simulink model "System_Modelled_SIMULINK"  (R2026a)
settings: Solver=VariableStepAuto  StopTime=3600
model workspace (MAT data in the model file):
  T_boot_threshold = 5
  T_overheat = 45
  T_storage_min = 8
  T_target = 15
libraries: fl_lib x12, nesl_utility x7, SignalEditorBlockLib x1

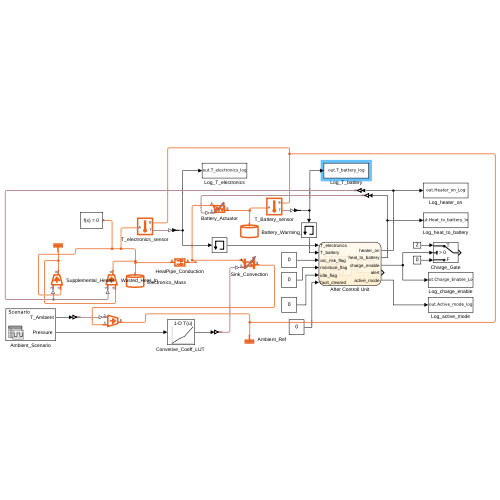
[thumbnail: Simulink's stored preview of the top-level diagram]
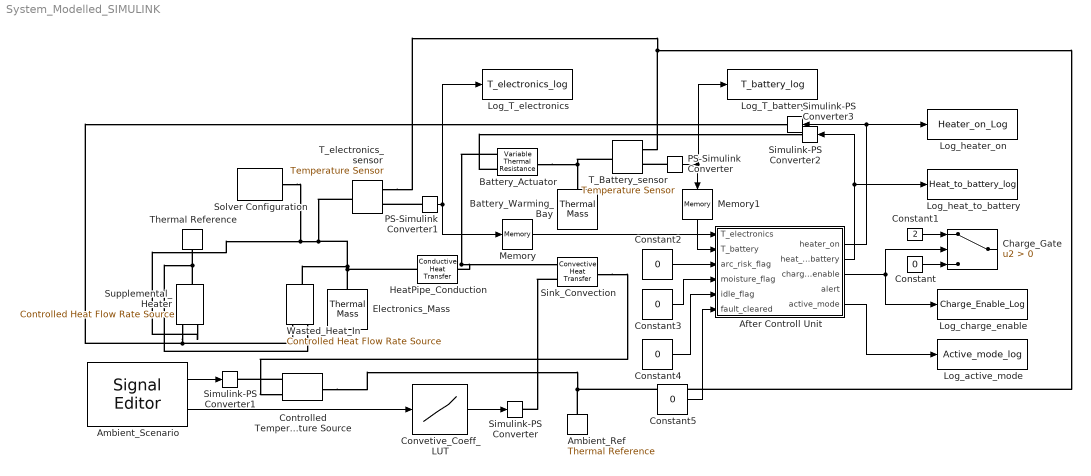
== system System_Modelled_SIMULINK ==
  After Controll Unit : Stateflow chart  TreatAsAtomicUnit=on
  Ambient_Ref : fl_lib/Thermal/Thermal Elements/Thermal Reference
  Ambient_Scenario : SignalEditorBlockLib/Signal Editor  FileName=/MATLAB Drive/SIH/Ambient_Scenario.mat  ActiveScenario=Scenario  ActiveSignal=T_Ambient  IsBus=off  OutputBusObjectStr=Bus: BusObject  SampleTime=0  ZeroCross=off  OutputAfterFinalValue=Setting to zero  Unit=inherit  PreserveSignalName=on  ApplySigPropsToAllScenarios=on  ApplySigPropsToAllSignals=off  SignalPropertySource=Dialog parameters
  Battery_Actuator : fl_lib/Thermal/Thermal Elements/Variable Thermal Resistance  R_min=0 K/W  T_specify=off  T_priority=None  T=0 K  T_nominal_specify=off  T_nominal_value=1  T_nominal_unit=K  Q_specify=off  Q_priority=None  Q=0 W  Q_nominal_specify=off  Q_nominal_value=1  Q_nominal_unit=W
  Battery_Warming_Bay : fl_lib/Thermal/Thermal Elements/Thermal Mass  mass_type=foundation.enum.constant_variable.constant  mass=1 kg  sp_heat=1000 J/(K*kg)  mass_min=1e-6 kg  num_ports=foundation.enum.numPorts2.one  m_specify=off  m_priority=High  m=1 kg  m_nominal_specify=off  m_nominal_value=1  m_nominal_unit=kg  T_specify=off  T_priority=High  T=300 K  T_nominal_specify=off  T_nominal_value=1  T_nominal_unit=K  Q_specify=off  Q_priority=None  Q=0 W  Q_nominal_specify=off  Q_nominal_value=1  Q_nominal_unit=W
  Charge_Gate : Switch  Criteria=u2 > Threshold  SaturateOnIntegerOverflow=off  InputSameDT=off
  Constant{,2..5} (5 alike) : Constant  Value=0
  Constant1 : Constant  Value=2
  Controlled Temperature Source : fl_lib/Thermal/Thermal Sources/Controlled Temperature Source
  "Convetive_Coeff_LUT " : Lookup_n-D  NumberOfTableDimensions=1  BreakpointsForDimension1=[50 60 70 80 101.3]  Table=[3 4 5 6 10]  InternalRulePriority=Speed  RndMeth=Simplest
  Electronics_Mass : fl_lib/Thermal/Thermal Elements/Thermal Mass  mass_type=foundation.enum.constant_variable.constant  mass=3 kg  sp_heat=900 J/(K*kg)  mass_min=1e-6 kg  num_ports=foundation.enum.numPorts2.one  m_specify=off  m_priority=High  m=1 kg  m_nominal_specify=off  m_nominal_value=1  m_nominal_unit=kg  T_specify=off  T_priority=High  T=300 K  T_nominal_specify=off  T_nominal_value=1  T_nominal_unit=K  Q_specify=off  Q_priority=None  Q=0 W  Q_nominal_specify=off  Q_nominal_value=1  Q_nominal_unit=W
  HeatPipe_Conduction : fl_lib/Thermal/Thermal Elements/Conductive Heat Transfer  thermal_type=foundation.enum.ConstantVariableTabulated.Constant  wall_geometry=foundation.enum.ConductionWallGeometry.Planar  area=5e-4 m^2  thickness=5e-3 m  d_in=0.05 m  d_out=0.1 m  L=1 m  th_cond_min=10 W/(K*m)  th_cond=2000 W/(K*m)  th_cond_TLU=[413, 401, 392, 383, 371, 357, 342] W/(K*m)  temp_TLU=[200, 273, 400, 600, 800, 1000, 1200] K  T_specify=off  T_priority=None  T=0 K  T_nominal_specify=off  T_nominal_value=1  T_nominal_unit=K  Q_specify=off  Q_priority=None  Q=0 W  Q_nominal_specify=off  Q_nominal_value=1  Q_nominal_unit=W
  Log_T_battery : ToWorkspace  VariableName=T_battery_log  SaveFormat=Timeseries  SampleTime=-1
  Log_T_electronics : ToWorkspace  VariableName=T_electronics_log  SaveFormat=Timeseries  SampleTime=-1
  Log_active_mode : ToWorkspace  VariableName=Active_mode_log  SaveFormat=Timeseries  SampleTime=-1
  Log_charge_enable : ToWorkspace  VariableName=Charge_Enable_Log  SaveFormat=Timeseries  SampleTime=-1
  Log_heat_to_battery : ToWorkspace  VariableName=Heat_to_battery_log  SaveFormat=Timeseries  SampleTime=-1
  Log_heater_on : ToWorkspace  VariableName=Heater_on_Log  SaveFormat=Timeseries  SampleTime=-1
  Memory : Memory
  Memory1 : Memory
  PS-Simulink Converter : nesl_utility/PS-Simulink Converter  PhysicalDomain=network_engine_domain  SubClassName=ps_output  LeftPortType=input  RightPortType=output  PseudoPeriodic=off  Frequencies=[]  VectorFormat=inherit  Unit=inherit  AffineConversion=off
  PS-Simulink Converter1 : nesl_utility/PS-Simulink Converter  PhysicalDomain=network_engine_domain  SubClassName=ps_output  LeftPortType=input  RightPortType=output  PseudoPeriodic=off  Frequencies=[]  VectorFormat=inherit  Unit=inherit  AffineConversion=off
  Simulink-PS Converter{,1..3} (4 alike) : nesl_utility/Simulink-PS Converter  PhysicalDomain=network_engine_domain  SubClassName=ps_input  LeftPortType=input  RightPortType=output  PseudoPeriodic=off  Frequencies=[]  NoiseDistribution=none  NoiseParameters=[]  Unit=1  AffineConversion=off  FilteringAndDerivatives=provide  SimscapeFilterOrder=1  InputFilterTimeConstant=0.001  UdotUserProvided=0
  Sink_Convection : fl_lib/Thermal/Thermal Elements/Convective Heat Transfer  thermal_type=foundation.enum.constant_variable.variable  area=1e-4 m^2  heat_tr_coeff=10 W/(K*m^2)  min_heat_tr_coeff=1e-3 W/(K*m^2)  T_specify=off  T_priority=None  T=0 K  T_nominal_specify=off  T_nominal_value=1  T_nominal_unit=K  Q_specify=off  Q_priority=None  Q=0 W  Q_nominal_specify=off  Q_nominal_value=1  Q_nominal_unit=W
  Solver Configuration : nesl_utility/Solver Configuration  PhysicalDomain=network_engine_domain  SubClassName=solver  LeftPortType=input  RightPortType=generic  Tones=[]  Harmonics=[]  SimulateNoise=off  Profile=off  UseLocalSampling=off  EnableSwitchedLinearOptims=on  FrequencyDomain=off  UseCCode=off  RelTol=0.001  AbsTol=0.001  MinStep=1e-09  ToWorkspace=off  RevertToSquareIcSolve=off  NumHomotopyIterations=100  PhasorMode=off  PhasorModeNumHarmonics=1  ConsistencySolver=NEWTON_XTOL_AFTER_FTOL  CanonicalOrdering=CANONICAL  OptimizeIntermediates=OPTIMIZED  IndexReductionMethod=DerivativeReplacement  DoDC=off  ResidualTolerance=1e-09  ConsistencyTolSource=GLOBAL  ConsistencyAbsTol=0.001  ConsistencyRelTol=0.001  ConsistencyTolFactor=0.001  UseLocalSolver=off  LocalSolverChoice=NE_BACKWARD_EULER_ADVANCER  ResolveIndetEquations=on  FunctionEvalNumThread=1  LocalSolverSampleTime=0.001  DoFixedCost=off  MaxNonlinIter=3  MaxModeIter=2  ComputeImpulses=off  ImpulseIterations=2  LinearAlgebra=auto  LinearAlgebraNumThread=0  EquationFormulation=NE_TIME_EF  DelaysMemoryBudget=1024  AutomaticFiltering=on  FilteringTimeConstant=0.001  PartitionStorageMethod=AS_NEEDED  PartitionMemoryBudget=1024  PartitionMethod=ROBUST  MultibodyUseLocalSolver=off  MultibodyLocalSolverChoice=ODE1  MultibodyLocalSolverSampleTime=0.001
  Supplemental_Heater : fl_lib/Thermal/Thermal Sources/Controlled Heat Flow Rate Source
  T_Battery_sensor : fl_lib/Thermal/Thermal Sensors/Temperature Sensor  temperature_measure=foundation.enum.MeasurementReference.difference
  T_electronics_sensor : fl_lib/Thermal/Thermal Sensors/Temperature Sensor  temperature_measure=foundation.enum.MeasurementReference.difference
  Thermal Reference : fl_lib/Thermal/Thermal Elements/Thermal Reference
  Wasted_Heat_In : fl_lib/Thermal/Thermal Sources/Controlled Heat Flow Rate Source
  wires:
  Constant1/1 -> Charge_Gate/1
  Constant/1 -> Charge_Gate/3
  After Controll Unit/3(charge_enable) -> Charge_Gate/2, Log_charge_enable/1
  Ambient_Scenario/1 -> Simulink-PS Converter1/1
  "Convetive_Coeff_LUT "/1 -> Simulink-PS Converter/1
  Ambient_Scenario/2 -> "Convetive_Coeff_LUT "/1
  PS-Simulink Converter/1 -> Memory1/1, Log_T_battery/1
  After Controll Unit/1(heater_on) -> Log_heater_on/1, Simulink-PS Converter2/1
  After Controll Unit/2(heat_to_battery) -> Simulink-PS Converter3/1, Log_heat_to_battery/1
  Constant2/1 -> After Controll Unit/3(arc_risk_flag)
  Constant3/1 -> After Controll Unit/4(moisture_flag)
  Constant4/1 -> After Controll Unit/5(idle_flag)
  Constant5/1 -> After Controll Unit/6(fault_cleared)
  After Controll Unit/5(active_mode) -> Log_active_mode/1
  PS-Simulink Converter1/1 -> Log_T_electronics/1, Memory/1
  Memory/1 -> After Controll Unit/1(T_electronics)
  Memory1/1 -> After Controll Unit/2(T_battery)
  connections:
  Electronics_Mass/LConn1 -- Wasted_Heat_In/LConn1 -- Supplemental_Heater/RConn2 -- Solver Configuration/RConn1 -- T_electronics_sensor/LConn1 -- HeatPipe_Conduction/LConn1
  Sink_Convection/LConn2 -- Simulink-PS Converter/RConn1
  Controlled Temperature Source/RConn1 -- Simulink-PS Converter1/RConn1
  Battery_Actuator/RConn1 -- T_Battery_sensor/LConn1 -- Battery_Warming_Bay/LConn1
  PS-Simulink Converter/LConn1 -- T_Battery_sensor/RConn2
  PS-Simulink Converter1/LConn1 -- T_electronics_sensor/RConn2
  Supplemental_Heater/RConn1 -- Simulink-PS Converter2/RConn1 -- Wasted_Heat_In/RConn1
  Battery_Actuator/LConn2 -- Simulink-PS Converter3/RConn1
  Ambient_Ref/LConn1 -- Controlled Temperature Source/LConn1 -- T_Battery_sensor/RConn1 -- T_electronics_sensor/RConn1
  Battery_Actuator/LConn1 -- Sink_Convection/LConn1 -- HeatPipe_Conduction/RConn1
  Supplemental_Heater/LConn1 -- Wasted_Heat_In/RConn2 -- Thermal Reference/LConn1
  Sink_Convection/RConn1 -- Controlled Temperature Source/RConn2

== stateflow chart System_Modelled_SIMULINK/After Controll Unit ==
  state SAFE
    state COLD_START
      entry: heater_on = 1; heat_to_battery = 0;
      charge_enable = 0; active_mode = 0;
    state NORMAL
      entry: heater_on = 0; active_mode = 1;
      during: heat_to_battery = double(T_battery < T_target);
      charge_enable = double(T_battery > 0);
    state STORAGE
      entry: active_mode = 2;
      during: heat_to_battery = double(T_battery < T_storage_min);
      charge_enable = double(T_battery > 0);
    SAFE -> COLD_START [order 1]
    (default) -> COLD_START
    COLD_START -> NORMAL : [T_electronics > T_boot_threshold]
    NORMAL -> STORAGE : [idle_flag == 1]
    STORAGE -> NORMAL : [idle_flag == 0]
  state FAULT
    entry: heat_to_battery = 0; heater_on = 0;
    charge_enable = 0; alert = 1; active_mode = 3;
  (default) -> SAFE
  SAFE -> FAULT [order 1] : [T_electronics > T_overheat || arc_risk_flag || moisture_flag]
  FAULT -> SAFE : [fault_cleared == 1]
  data: T_electronics input double size=1; T_battery input double size=1; arc_risk_flag input double size=1; moisture_flag input double size=1; idle_flag input double size=1; fault_cleared input double size=1; T_boot_threshold parameter double; T_target parameter double; T_storage_min parameter double; heater_on output size=1; heat_to_battery output size=1; charge_enable output size=1; alert output size=1; active_mode output size=1; T_overheat parameter double
